simulink model "pfb_fft_d3a"  (R2021a)
settings: Solver=VariableStepAuto  StartTime=0.0  StopTime=100.0  RelTol=1e-3
undefined symbols (not defined in the file): i, pfb_coeff_gen_calc
libraries: xbsIndex_r4 x11529, casper_library_misc x39, casper_library_delays x39, xbsReplacements_r4 x2
(part 52 of 118)

== system pfb_fft_d3a/fft_wideband_real/fft_direct/butterfly2_0/bus_scale/bussify ==
  in1 : Inport
  in2 : Inport  Port=2
  in3 : Inport  Port=3
  in4 : Inport  Port=4
  concatenate : xbsIndex_r4/Concat  num_inputs=4  dbl_ovrd=off  block_type=concat
  reinterpret{1..4} (4 alike) : xbsIndex_r4/Reinterpret  force_arith_type=on  arith_type=Unsigned  force_bin_pt=on  bin_pt=0  block_type=reinterpret
      reinterpret1 settings: infoedit="Changes signal type without altering the binary representation.   You can changed the signal between signed and unsigned, and relocate the binary point.<br><br>Hardware notes: In hardware this block costs nothing.<br><br>Example:  Suppose the input is 6 bits wide, signed, with 2 fractional bits, and the output is forced to unsigned with 0 fractional bits.  Then an input of -2.0 (1110.00 in binary 2's complement) becomes an output of 56 (111000 in binary)."
      reinterpret2 settings: infoedit="Changes signal type without altering the binary representation.   You can changed the signal between signed and unsigned, and relocate the binary point.<br><br>Hardware notes: In hardware this block costs nothing.<br><br>Example:  Suppose the input is 6 bits wide, signed, with 2 fractional bits, and the output is forced to unsigned with 0 fractional bits.  Then an input of -2.0 (1110.00 in binary 2's complement) becomes an output of 56 (111000 in binary)."
  bus_out : Outport  VectorParamsAs1DForOutWhenUnconnected=off
  wires:
  concatenate/1 -> bus_out/1
  in1/1 -> reinterpret1/1
  reinterpret1/1 -> concatenate/1
  in2/1 -> reinterpret2/1
  reinterpret2/1 -> concatenate/2
  in3/1 -> reinterpret3/1
  reinterpret3/1 -> concatenate/3
  in4/1 -> reinterpret4/1
  reinterpret4/1 -> concatenate/4

== system pfb_fft_d3a/fft_wideband_real/fft_direct/butterfly2_0/bus_scale/debus ==
  bus_in : Inport
  reinterpret{1..4} (4 alike) : xbsIndex_r4/Reinterpret  force_arith_type=on  arith_type="Signed  (2's comp)"  force_bin_pt=on  bin_pt=17  block_type=reinterpret
  slice1 : xbsIndex_r4/Slice  nbits=20  boolean_output=off  mode=Upper Bit Location + Width  bit1=-60  base1=MSB of Input  bit0=0  base0=LSB of Input  dbl_ovrd=off  block_type=slice
  slice2 : xbsIndex_r4/Slice  nbits=20  boolean_output=off  mode=Upper Bit Location + Width  bit1=-40  base1=MSB of Input  bit0=0  base0=LSB of Input  dbl_ovrd=off  block_type=slice
  slice3 : xbsIndex_r4/Slice  nbits=20  boolean_output=off  mode=Upper Bit Location + Width  bit1=-20  base1=MSB of Input  bit0=0  base0=LSB of Input  dbl_ovrd=off  block_type=slice
  slice4 : xbsIndex_r4/Slice  nbits=20  boolean_output=off  mode=Upper Bit Location + Width  bit1=0  base1=MSB of Input  bit0=0  base0=LSB of Input  dbl_ovrd=off  block_type=slice
  msb_out4 : Outport
  out3 : Outport  Port=2
  out2 : Outport  Port=3
  lsb_out1 : Outport  Port=4  VectorParamsAs1DForOutWhenUnconnected=off
  wires:
  bus_in/1 -> slice4/1, slice3/1, slice2/1, slice1/1
  slice4/1 -> reinterpret4/1
  reinterpret4/1 -> msb_out4/1
  slice3/1 -> reinterpret3/1
  reinterpret3/1 -> out3/1
  slice2/1 -> reinterpret2/1
  reinterpret2/1 -> out2/1
  slice1/1 -> reinterpret1/1
  reinterpret1/1 -> lsb_out1/1

== system pfb_fft_d3a/fft_wideband_real/fft_direct/butterfly2_0/bus_sub/a_debus ==
  bus_in : Inport
  reinterpret1 : xbsIndex_r4/Reinterpret  force_arith_type=on  arith_type="Signed  (2's comp)"  force_bin_pt=on  bin_pt=17  block_type=reinterpret
  reinterpret2 : xbsIndex_r4/Reinterpret  force_arith_type=on  arith_type="Signed  (2's comp)"  force_bin_pt=on  bin_pt=17  block_type=reinterpret
  slice1 : xbsIndex_r4/Slice  nbits=18  boolean_output=off  mode=Upper Bit Location + Width  bit1=-18  base1=MSB of Input  bit0=0  base0=LSB of Input  dbl_ovrd=off  block_type=slice
  slice2 : xbsIndex_r4/Slice  nbits=18  boolean_output=off  mode=Upper Bit Location + Width  bit1=0  base1=MSB of Input  bit0=0  base0=LSB of Input  dbl_ovrd=off  block_type=slice
  msb_out2 : Outport  VectorParamsAs1DForOutWhenUnconnected=off
  lsb_out1 : Outport  Port=2  VectorParamsAs1DForOutWhenUnconnected=off
  wires:
  bus_in/1 -> slice2/1, slice1/1
  slice2/1 -> reinterpret2/1
  reinterpret2/1 -> msb_out2/1
  slice1/1 -> reinterpret1/1
  reinterpret1/1 -> lsb_out1/1

== system pfb_fft_d3a/fft_wideband_real/fft_direct/butterfly2_0/bus_sub/b_debus ==
  bus_in : Inport
  reinterpret1 : xbsIndex_r4/Reinterpret  force_arith_type=on  arith_type="Signed  (2's comp)"  force_bin_pt=on  bin_pt=17  block_type=reinterpret
  reinterpret2 : xbsIndex_r4/Reinterpret  force_arith_type=on  arith_type="Signed  (2's comp)"  force_bin_pt=on  bin_pt=17  block_type=reinterpret
  slice1 : xbsIndex_r4/Slice  nbits=19  boolean_output=off  mode=Upper Bit Location + Width  bit1=-19  base1=MSB of Input  bit0=0  base0=LSB of Input  dbl_ovrd=off  block_type=slice
  slice2 : xbsIndex_r4/Slice  nbits=19  boolean_output=off  mode=Upper Bit Location + Width  bit1=0  base1=MSB of Input  bit0=0  base0=LSB of Input  dbl_ovrd=off  block_type=slice
  msb_out2 : Outport  VectorParamsAs1DForOutWhenUnconnected=off
  lsb_out1 : Outport  Port=2  VectorParamsAs1DForOutWhenUnconnected=off
  wires:
  bus_in/1 -> slice2/1, slice1/1
  slice2/1 -> reinterpret2/1
  reinterpret2/1 -> msb_out2/1
  slice1/1 -> reinterpret1/1
  reinterpret1/1 -> lsb_out1/1

== system pfb_fft_d3a/fft_wideband_real/fft_direct/butterfly2_0/bus_sub/op_bussify ==
  in1 : Inport
  in2 : Inport  Port=2
  concatenate : xbsIndex_r4/Concat  num_inputs=2  dbl_ovrd=off  block_type=concat
  reinterpret1 : xbsIndex_r4/Reinterpret  force_arith_type=on  arith_type=Unsigned  force_bin_pt=on  bin_pt=0  block_type=reinterpret
      settings: infoedit="Changes signal type without altering the binary representation.   You can changed the signal between signed and unsigned, and relocate the binary point.<br><br>Hardware notes: In hardware this block costs nothing.<br><br>Example:  Suppose the input is 6 bits wide, signed, with 2 fractional bits, and the output is forced to unsigned with 0 fractional bits.  Then an input of -2.0 (1110.00 in binary 2's complement) becomes an output of 56 (111000 in binary)."
  reinterpret2 : xbsIndex_r4/Reinterpret  force_arith_type=on  arith_type=Unsigned  force_bin_pt=on  bin_pt=0  block_type=reinterpret
      settings: infoedit="Changes signal type without altering the binary representation.   You can changed the signal between signed and unsigned, and relocate the binary point.<br><br>Hardware notes: In hardware this block costs nothing.<br><br>Example:  Suppose the input is 6 bits wide, signed, with 2 fractional bits, and the output is forced to unsigned with 0 fractional bits.  Then an input of -2.0 (1110.00 in binary 2's complement) becomes an output of 56 (111000 in binary)."
  bus_out : Outport  VectorParamsAs1DForOutWhenUnconnected=off
  wires:
  concatenate/1 -> bus_out/1
  in1/1 -> reinterpret1/1
  reinterpret1/1 -> concatenate/1
  in2/1 -> reinterpret2/1
  reinterpret2/1 -> concatenate/2

== system pfb_fft_d3a/fft_wideband_real/fft_direct/butterfly2_0/munge/join ==
  in1 : Inport
  in2 : Inport  Port=2
  concatenate : xbsIndex_r4/Concat  num_inputs=2  dbl_ovrd=off  block_type=concat
  reinterpret1 : xbsIndex_r4/Reinterpret  force_arith_type=on  arith_type=Unsigned  force_bin_pt=on  bin_pt=0  block_type=reinterpret
      settings: infoedit="Changes signal type without altering the binary representation.   You can changed the signal between signed and unsigned, and relocate the binary point.<br><br>Hardware notes: In hardware this block costs nothing.<br><br>Example:  Suppose the input is 6 bits wide, signed, with 2 fractional bits, and the output is forced to unsigned with 0 fractional bits.  Then an input of -2.0 (1110.00 in binary 2's complement) becomes an output of 56 (111000 in binary)."
  reinterpret2 : xbsIndex_r4/Reinterpret  force_arith_type=on  arith_type=Unsigned  force_bin_pt=on  bin_pt=0  block_type=reinterpret
      settings: infoedit="Changes signal type without altering the binary representation.   You can changed the signal between signed and unsigned, and relocate the binary point.<br><br>Hardware notes: In hardware this block costs nothing.<br><br>Example:  Suppose the input is 6 bits wide, signed, with 2 fractional bits, and the output is forced to unsigned with 0 fractional bits.  Then an input of -2.0 (1110.00 in binary 2's complement) becomes an output of 56 (111000 in binary)."
  bus_out : Outport  VectorParamsAs1DForOutWhenUnconnected=off
  wires:
  concatenate/1 -> bus_out/1
  in1/1 -> reinterpret1/1
  reinterpret1/1 -> concatenate/1
  in2/1 -> reinterpret2/1
  reinterpret2/1 -> concatenate/2

== system pfb_fft_d3a/fft_wideband_real/fft_direct/butterfly2_0/munge/split ==
  bus_in : Inport
  reinterpret1 : xbsIndex_r4/Reinterpret  force_arith_type=on  arith_type=Unsigned  force_bin_pt=on  bin_pt=0  block_type=reinterpret
  reinterpret2 : xbsIndex_r4/Reinterpret  force_arith_type=on  arith_type=Unsigned  force_bin_pt=on  bin_pt=0  block_type=reinterpret
  slice1 : xbsIndex_r4/Slice  nbits=2  boolean_output=off  mode=Upper Bit Location + Width  bit1=-2  base1=MSB of Input  bit0=0  base0=LSB of Input  dbl_ovrd=off  block_type=slice
  slice2 : xbsIndex_r4/Slice  nbits=2  boolean_output=off  mode=Upper Bit Location + Width  bit1=0  base1=MSB of Input  bit0=0  base0=LSB of Input  dbl_ovrd=off  block_type=slice
  msb_out2 : Outport  VectorParamsAs1DForOutWhenUnconnected=off
  lsb_out1 : Outport  Port=2  VectorParamsAs1DForOutWhenUnconnected=off
  wires:
  bus_in/1 -> slice2/1, slice1/1
  slice2/1 -> reinterpret2/1
  reinterpret2/1 -> msb_out2/1
  slice1/1 -> reinterpret1/1
  reinterpret1/1 -> lsb_out1/1

== system pfb_fft_d3a/fft_wideband_real/fft_direct/butterfly2_0/mux/d_bussify ==
  in1 : Inport
  in2 : Inport  Port=2
  in3 : Inport  Port=3
  in4 : Inport  Port=4
  concatenate : xbsIndex_r4/Concat  num_inputs=4  dbl_ovrd=off  block_type=concat
  reinterpret{1..4} (4 alike) : xbsIndex_r4/Reinterpret  force_arith_type=on  arith_type=Unsigned  force_bin_pt=on  bin_pt=0  block_type=reinterpret
      reinterpret1 settings: infoedit="Changes signal type without altering the binary representation.   You can changed the signal between signed and unsigned, and relocate the binary point.<br><br>Hardware notes: In hardware this block costs nothing.<br><br>Example:  Suppose the input is 6 bits wide, signed, with 2 fractional bits, and the output is forced to unsigned with 0 fractional bits.  Then an input of -2.0 (1110.00 in binary 2's complement) becomes an output of 56 (111000 in binary)."
      reinterpret2 settings: infoedit="Changes signal type without altering the binary representation.   You can changed the signal between signed and unsigned, and relocate the binary point.<br><br>Hardware notes: In hardware this block costs nothing.<br><br>Example:  Suppose the input is 6 bits wide, signed, with 2 fractional bits, and the output is forced to unsigned with 0 fractional bits.  Then an input of -2.0 (1110.00 in binary 2's complement) becomes an output of 56 (111000 in binary)."
  bus_out : Outport  VectorParamsAs1DForOutWhenUnconnected=off
  wires:
  concatenate/1 -> bus_out/1
  in1/1 -> reinterpret1/1
  reinterpret1/1 -> concatenate/1
  in2/1 -> reinterpret2/1
  reinterpret2/1 -> concatenate/2
  in3/1 -> reinterpret3/1
  reinterpret3/1 -> concatenate/3
  in4/1 -> reinterpret4/1
  reinterpret4/1 -> concatenate/4

== system pfb_fft_d3a/fft_wideband_real/fft_direct/butterfly2_0/mux/expand0 ==
  bus_in : Inport
  reinterpret{1..4} (4 alike) : xbsIndex_r4/Reinterpret  force_arith_type=on  arith_type=Unsigned  force_bin_pt=on  bin_pt=0  block_type=reinterpret
  slice1 : xbsIndex_r4/Slice  nbits=21  boolean_output=off  mode=Upper Bit Location + Width  bit1=-63  base1=MSB of Input  bit0=0  base0=LSB of Input  dbl_ovrd=off  block_type=slice
  slice2 : xbsIndex_r4/Slice  nbits=21  boolean_output=off  mode=Upper Bit Location + Width  bit1=-42  base1=MSB of Input  bit0=0  base0=LSB of Input  dbl_ovrd=off  block_type=slice
  slice3 : xbsIndex_r4/Slice  nbits=21  boolean_output=off  mode=Upper Bit Location + Width  bit1=-21  base1=MSB of Input  bit0=0  base0=LSB of Input  dbl_ovrd=off  block_type=slice
  slice4 : xbsIndex_r4/Slice  nbits=21  boolean_output=off  mode=Upper Bit Location + Width  bit1=0  base1=MSB of Input  bit0=0  base0=LSB of Input  dbl_ovrd=off  block_type=slice
  msb_out4 : Outport
  out3 : Outport  Port=2
  out2 : Outport  Port=3
  lsb_out1 : Outport  Port=4  VectorParamsAs1DForOutWhenUnconnected=off
  wires:
  bus_in/1 -> slice4/1, slice3/1, slice2/1, slice1/1
  slice4/1 -> reinterpret4/1
  reinterpret4/1 -> msb_out4/1
  slice3/1 -> reinterpret3/1
  reinterpret3/1 -> out3/1
  slice2/1 -> reinterpret2/1
  reinterpret2/1 -> out2/1
  slice1/1 -> reinterpret1/1
  reinterpret1/1 -> lsb_out1/1

== system pfb_fft_d3a/fft_wideband_real/fft_direct/butterfly2_0/mux/expand1 ==
  bus_in : Inport
  reinterpret{1..4} (4 alike) : xbsIndex_r4/Reinterpret  force_arith_type=on  arith_type=Unsigned  force_bin_pt=on  bin_pt=0  block_type=reinterpret
  slice1 : xbsIndex_r4/Slice  nbits=21  boolean_output=off  mode=Upper Bit Location + Width  bit1=-63  base1=MSB of Input  bit0=0  base0=LSB of Input  dbl_ovrd=off  block_type=slice
  slice2 : xbsIndex_r4/Slice  nbits=21  boolean_output=off  mode=Upper Bit Location + Width  bit1=-42  base1=MSB of Input  bit0=0  base0=LSB of Input  dbl_ovrd=off  block_type=slice
  slice3 : xbsIndex_r4/Slice  nbits=21  boolean_output=off  mode=Upper Bit Location + Width  bit1=-21  base1=MSB of Input  bit0=0  base0=LSB of Input  dbl_ovrd=off  block_type=slice
  slice4 : xbsIndex_r4/Slice  nbits=21  boolean_output=off  mode=Upper Bit Location + Width  bit1=0  base1=MSB of Input  bit0=0  base0=LSB of Input  dbl_ovrd=off  block_type=slice
  msb_out4 : Outport
  out3 : Outport  Port=2
  out2 : Outport  Port=3
  lsb_out1 : Outport  Port=4  VectorParamsAs1DForOutWhenUnconnected=off
  wires:
  bus_in/1 -> slice4/1, slice3/1, slice2/1, slice1/1
  slice4/1 -> reinterpret4/1
  reinterpret4/1 -> msb_out4/1
  slice3/1 -> reinterpret3/1
  reinterpret3/1 -> out3/1
  slice2/1 -> reinterpret2/1
  reinterpret2/1 -> out2/1
  slice1/1 -> reinterpret1/1
  reinterpret1/1 -> lsb_out1/1

== system pfb_fft_d3a/fft_wideband_real/fft_direct/butterfly2_0/mux/sel_expand ==
  bus_in : Inport
  reinterpret{1..4} (4 alike) : xbsIndex_r4/Reinterpret  force_arith_type=on  arith_type=Unsigned  force_bin_pt=on  bin_pt=0  block_type=reinterpret
  slice1 : xbsIndex_r4/Slice  nbits=1  boolean_output=off  mode=Upper Bit Location + Width  bit1=-3  base1=MSB of Input  bit0=0  base0=LSB of Input  dbl_ovrd=off  block_type=slice
  slice2 : xbsIndex_r4/Slice  nbits=1  boolean_output=off  mode=Upper Bit Location + Width  bit1=-2  base1=MSB of Input  bit0=0  base0=LSB of Input  dbl_ovrd=off  block_type=slice
  slice3 : xbsIndex_r4/Slice  nbits=1  boolean_output=off  mode=Upper Bit Location + Width  bit1=-1  base1=MSB of Input  bit0=0  base0=LSB of Input  dbl_ovrd=off  block_type=slice
  slice4 : xbsIndex_r4/Slice  nbits=1  boolean_output=off  mode=Upper Bit Location + Width  bit1=0  base1=MSB of Input  bit0=0  base0=LSB of Input  dbl_ovrd=off  block_type=slice
  msb_out4 : Outport
  out3 : Outport  Port=2
  out2 : Outport  Port=3
  lsb_out1 : Outport  Port=4  VectorParamsAs1DForOutWhenUnconnected=off
  wires:
  bus_in/1 -> slice4/1, slice3/1, slice2/1, slice1/1
  slice4/1 -> reinterpret4/1
  reinterpret4/1 -> msb_out4/1
  slice3/1 -> reinterpret3/1
  reinterpret3/1 -> out3/1
  slice2/1 -> reinterpret2/1
  reinterpret2/1 -> out2/1
  slice1/1 -> reinterpret1/1
  reinterpret1/1 -> lsb_out1/1

== system pfb_fft_d3a/fft_wideband_real/fft_direct/butterfly2_0/shift_replicate/bussify ==
  in1 : Inport
  in2 : Inport  Port=2
  in3 : Inport  Port=3
  in4 : Inport  Port=4
  concatenate : xbsIndex_r4/Concat  num_inputs=4  dbl_ovrd=off  block_type=concat
  reinterpret{1..4} (4 alike) : xbsIndex_r4/Reinterpret  force_arith_type=on  arith_type=Unsigned  force_bin_pt=on  bin_pt=0  block_type=reinterpret
      reinterpret1 settings: infoedit="Changes signal type without altering the binary representation.   You can changed the signal between signed and unsigned, and relocate the binary point.<br><br>Hardware notes: In hardware this block costs nothing.<br><br>Example:  Suppose the input is 6 bits wide, signed, with 2 fractional bits, and the output is forced to unsigned with 0 fractional bits.  Then an input of -2.0 (1110.00 in binary 2's complement) becomes an output of 56 (111000 in binary)."
      reinterpret2 settings: infoedit="Changes signal type without altering the binary representation.   You can changed the signal between signed and unsigned, and relocate the binary point.<br><br>Hardware notes: In hardware this block costs nothing.<br><br>Example:  Suppose the input is 6 bits wide, signed, with 2 fractional bits, and the output is forced to unsigned with 0 fractional bits.  Then an input of -2.0 (1110.00 in binary 2's complement) becomes an output of 56 (111000 in binary)."
  bus_out : Outport  VectorParamsAs1DForOutWhenUnconnected=off
  wires:
  concatenate/1 -> bus_out/1
  in1/1 -> reinterpret1/1
  reinterpret1/1 -> concatenate/1
  in2/1 -> reinterpret2/1
  reinterpret2/1 -> concatenate/2
  in3/1 -> reinterpret3/1
  reinterpret3/1 -> concatenate/3
  in4/1 -> reinterpret4/1
  reinterpret4/1 -> concatenate/4

== system pfb_fft_d3a/fft_wideband_real/fft_direct/butterfly2_0/twiddle/bus_convert ==
  din : Inport
  misci : Inport  Port=2
  bussify : Subsystem  AncestorBlock=casper_library_flow_control/bus_create  mask(bus_create){inputNum=2}
      mask prompts: inputNum "Number of inputs:"
      mask init:
      | bus_create_init(gcb,...
      |     'inputNum', inputNum);
  conv1 : xbsIndex_r4/Convert  gui_display_data_type=Fixed-point  arith_type="Signed  (2's comp)"  n_bits=19  bin_pt=17  float_type=Single  exp_bits=8  fraction_bits=24  quantization="Round  (unbiased: Even Values)"  overflow=Wrap  en=off  latency=1  pipeline=on  dbl_ovrd=off  block_type=convert
  conv2 : xbsIndex_r4/Convert  gui_display_data_type=Fixed-point  arith_type="Signed  (2's comp)"  n_bits=19  bin_pt=17  float_type=Single  exp_bits=8  fraction_bits=24  quantization="Round  (unbiased: Even Values)"  overflow=Wrap  en=off  latency=1  pipeline=on  dbl_ovrd=off  block_type=convert
  debus : Subsystem  AncestorBlock=casper_library_flow_control/bus_expand  mask(bus_expand){mode=divisions of arbitrary size, outputNum=2, outputWidth=[37 37], outputBinaryPt=[34 34], outputArithmeticType=[1 1], show_format=on, outputToWorkspace=off, variablePrefix=, outputToModelAsWell=on}
      mask prompts: outputNum "Number of outputs:"; outputWidth "Output width:"; outputBinaryPt "Output binary point position:"; outputArithmeticType "Output arithmetic type (ufix=0, fix=1, bool=2):"; show_format "Print format string?"; outputToWorkspace "Output to workspace?"; variablePrefix "Variable name prefix:"; outputToModelAsWell "Output to model as well?"
      mask help:
      | Expands a 'bus' made using a bus_create or Xilinx
      | concat block.
      | The input will be divided into the specified number
      | of outputs with the specified arithmetic types.
      | Divisions are made from most significant bit.
      mask init: same as pfb_fft_d3a/fft_wideband_real/fft_biplex_real_4x/pol0_debus
      settings: AttributesFormatString=2 outputs: f37.34,f37.34,
      mask TypeOptions mode: divisions of equal size | divisions of arbitrary size
      mask Callback mode: %bus_expand_callback();
      mask Callback outputWidth: %bus_expand_callback();
      mask Callback outputToWorkspace: %bus_expand_callback();
  dmisc : xbsIndex_r4/Delay  rst=off  infoeditControl=Selection of Reset will increase slice count due to use of real FFs and instead of SRLs  en=off  latency=csp_latency  reg_retiming=on  dbl_ovrd=off  block_type=delay
  dout : Outport
  misco : Outport  Port=2
  wires:
  din/1 -> debus/1(bus_in)
  debus/1(msb_out2) -> conv1/1
  debus/2(lsb_out1) -> conv2/1
  misci/1 -> dmisc/1
  conv1/1 -> bussify/1(in1)
  conv2/1 -> bussify/2(in2)
  bussify/1(bus_out) -> dout/1
  dmisc/1 -> misco/1

== system pfb_fft_d3a/fft_wideband_real/fft_direct/butterfly2_0/twiddle/bus_create ==
  in1 : Inport
  in2 : Inport  Port=2
  in3 : Inport  Port=3
  concatenate : xbsIndex_r4/Concat  num_inputs=3  dbl_ovrd=off  block_type=concat
  reinterpret1 : xbsIndex_r4/Reinterpret  force_arith_type=on  arith_type=Unsigned  force_bin_pt=on  bin_pt=0  block_type=reinterpret
      settings: infoedit="Changes signal type without altering the binary representation.   You can changed the signal between signed and unsigned, and relocate the binary point.<br><br>Hardware notes: In hardware this block costs nothing.<br><br>Example:  Suppose the input is 6 bits wide, signed, with 2 fractional bits, and the output is forced to unsigned with 0 fractional bits.  Then an input of -2.0 (1110.00 in binary 2's complement) becomes an output of 56 (111000 in binary)."
  reinterpret2 : xbsIndex_r4/Reinterpret  force_arith_type=on  arith_type=Unsigned  force_bin_pt=on  bin_pt=0  block_type=reinterpret
      settings: infoedit="Changes signal type without altering the binary representation.   You can changed the signal between signed and unsigned, and relocate the binary point.<br><br>Hardware notes: In hardware this block costs nothing.<br><br>Example:  Suppose the input is 6 bits wide, signed, with 2 fractional bits, and the output is forced to unsigned with 0 fractional bits.  Then an input of -2.0 (1110.00 in binary 2's complement) becomes an output of 56 (111000 in binary)."
  reinterpret3 : xbsIndex_r4/Reinterpret  force_arith_type=on  arith_type=Unsigned  force_bin_pt=on  bin_pt=0  block_type=reinterpret
  bus_out : Outport  VectorParamsAs1DForOutWhenUnconnected=off
  wires:
  concatenate/1 -> bus_out/1
  in1/1 -> reinterpret1/1
  reinterpret1/1 -> concatenate/1
  in2/1 -> reinterpret2/1
  reinterpret2/1 -> concatenate/2
  in3/1 -> reinterpret3/1
  reinterpret3/1 -> concatenate/3

== system pfb_fft_d3a/fft_wideband_real/fft_direct/butterfly2_0/twiddle/bus_expand ==
  bus_in : Inport
  reinterpret1 : xbsIndex_r4/Reinterpret  force_arith_type=on  arith_type=Unsigned  force_bin_pt=on  bin_pt=0  block_type=reinterpret
  reinterpret2 : xbsIndex_r4/Reinterpret  force_arith_type=on  arith_type=Unsigned  force_bin_pt=on  bin_pt=0  block_type=reinterpret
  slice1 : xbsIndex_r4/Slice  nbits=37  boolean_output=off  mode=Upper Bit Location + Width  bit1=-36  base1=MSB of Input  bit0=0  base0=LSB of Input  dbl_ovrd=off  block_type=slice
  slice2 : xbsIndex_r4/Slice  nbits=36  boolean_output=off  mode=Upper Bit Location + Width  bit1=0  base1=MSB of Input  bit0=0  base0=LSB of Input  dbl_ovrd=off  block_type=slice
  msb_out2 : Outport  VectorParamsAs1DForOutWhenUnconnected=off
  lsb_out1 : Outport  Port=2  VectorParamsAs1DForOutWhenUnconnected=off
  wires:
  bus_in/1 -> slice2/1, slice1/1
  slice2/1 -> reinterpret2/1
  reinterpret2/1 -> msb_out2/1
  slice1/1 -> reinterpret1/1
  reinterpret1/1 -> lsb_out1/1

== system pfb_fft_d3a/fft_wideband_real/fft_direct/butterfly2_0/twiddle/bus_expand1 ==
  bus_in : Inport
  reinterpret1 : xbsIndex_r4/Reinterpret  force_arith_type=on  arith_type=Unsigned  force_bin_pt=on  bin_pt=0  block_type=reinterpret
  slice1 : xbsIndex_r4/Slice  nbits=36  boolean_output=off  mode=Upper Bit Location + Width  bit1=-1  base1=MSB of Input  bit0=0  base0=LSB of Input  dbl_ovrd=off  block_type=slice
  slice2 : xbsIndex_r4/Slice  nbits=1  boolean_output=on  mode=Upper Bit Location + Width  bit1=0  base1=MSB of Input  bit0=0  base0=LSB of Input  dbl_ovrd=off  block_type=slice
  msb_out2 : Outport  VectorParamsAs1DForOutWhenUnconnected=off
  lsb_out1 : Outport  Port=2  VectorParamsAs1DForOutWhenUnconnected=off
  wires:
  bus_in/1 -> slice2/1, slice1/1
  slice2/1 -> msb_out2/1
  slice1/1 -> reinterpret1/1
  reinterpret1/1 -> lsb_out1/1

== system pfb_fft_d3a/fft_wideband_real/fft_direct/butterfly2_0/twiddle/bus_mult ==
  a : Inport
  b : Inport  Port=2
  misci : Inport  Port=3
  a*b_bussify : Subsystem  AncestorBlock=casper_library_flow_control/bus_create  mask(bus_create){inputNum=1}
      mask prompts: inputNum "Number of inputs:"
      mask init:
      | bus_create_init(gcb,...
      |     'inputNum', inputNum);
  a_debus : Subsystem  AncestorBlock=casper_library_flow_control/bus_expand  mask(bus_expand){mode=divisions of arbitrary size, outputNum=2, outputWidth=36, outputBinaryPt=0, outputArithmeticType=0, show_format=on, outputToWorkspace=off, variablePrefix=, outputToModelAsWell=on}
      mask prompts: outputNum "Number of outputs:"; outputWidth "Output width:"; outputBinaryPt "Output binary point position:"; outputArithmeticType "Output arithmetic type (ufix=0, fix=1, bool=2):"; show_format "Print format string?"; outputToWorkspace "Output to workspace?"; variablePrefix "Variable name prefix:"; outputToModelAsWell "Output to model as well?"
      mask help:
      | Expands a 'bus' made using a bus_create or Xilinx
      | concat block.
      | The input will be divided into the specified number
      | of outputs with the specified arithmetic types.
      | Divisions are made from most significant bit.
      mask init: same as pfb_fft_d3a/fft_wideband_real/fft_biplex_real_4x/pol0_debus
      settings: AttributesFormatString=1 outputs: uf36.0,
      mask TypeOptions mode: divisions of equal size | divisions of arbitrary size
      mask Callback mode: %bus_expand_callback();
      mask Callback outputWidth: %bus_expand_callback();
      mask Callback outputToWorkspace: %bus_expand_callback();
  b_debus : Subsystem  AncestorBlock=casper_library_flow_control/bus_expand  mask(bus_expand){mode=divisions of arbitrary size, outputNum=2, outputWidth=36, outputBinaryPt=0, outputArithmeticType=0, show_format=on, outputToWorkspace=off, variablePrefix=, outputToModelAsWell=on}
      mask prompts: outputNum "Number of outputs:"; outputWidth "Output width:"; outputBinaryPt "Output binary point position:"; outputArithmeticType "Output arithmetic type (ufix=0, fix=1, bool=2):"; show_format "Print format string?"; outputToWorkspace "Output to workspace?"; variablePrefix "Variable name prefix:"; outputToModelAsWell "Output to model as well?"
      mask help:
      | Expands a 'bus' made using a bus_create or Xilinx
      | concat block.
      | The input will be divided into the specified number
      | of outputs with the specified arithmetic types.
      | Divisions are made from most significant bit.
      mask init: same as pfb_fft_d3a/fft_wideband_real/fft_biplex_real_4x/pol0_debus
      settings: AttributesFormatString=1 outputs: uf36.0,
      mask TypeOptions mode: divisions of equal size | divisions of arbitrary size
      mask Callback mode: %bus_expand_callback();
      mask Callback outputWidth: %bus_expand_callback();
      mask Callback outputToWorkspace: %bus_expand_callback();
  dmisc : xbsIndex_r4/Delay  rst=off  infoeditControl=Selection of Reset will increase slice count due to use of real FFs and instead of SRLs  en=off  latency=mult_latency+add_latency+conv_latency+fan_latency  reg_retiming=on  dbl_ovrd=off  block_type=delay
  mult1 : Subsystem  AncestorBlock=casper_library_multipliers/cmult  mask(cmult){n_bits_a=18, bin_pt_a=17, n_bits_b=18, bin_pt_b=17, n_bits_ab=37, bin_pt_ab=34, quantization=Truncate, overflow=Wrap, conjugated=off, async=off, pipelined_enable=on, floating_point=off, float_type=single, exp_width=8, frac_width=24, in_latency=0, mult_latency=2, add_latency=1, conv_latency=0, pipeline_cmult_en=off, pipeline_latency=0, multiplier_implementation=behavioral HDL}
      mask prompts: n_bits_a "Number of Bits 'a'"; bin_pt_a "Binary Point 'a'"; n_bits_b "Number of Bits 'b'"; bin_pt_b "Binary Point 'b'"; n_bits_ab "Number of Bits 'ab'"; bin_pt_ab "Binary Point 'ab'"; conjugated "Conjugate"; async "asynchronous operation"; pipelined_enable "enable pipeline"; floating_point "floating point"; float_type "float type"; exp_width "exponent width"; frac_width "fraction width"; in_latency "Input latency"; mult_latency "Multiplier Latency"; add_latency "Adder Latency"; conv_latency "Convert latency"; pipeline_cmult_en "Pipeline cmult enable"; pipeline_latency "Pipeline latency"; multiplier_implementation "Multiplier implementation"
      mask help:
      | Multiplies two complex numbers using 4 multipliers and 2 adders.
      | Conjugation is optional.
      mask init: same as pfb_fft_d3a/fft_wideband_real/fft_direct/butterfly0_0/twiddle/bus_mult/mult1
      settings: AttributesFormatString=|
      | 18_17 * 18_17 ==> 37_34
      | Truncate, Wrap
      | Latency=0
      mask TypeOptions quantization: Truncate | Round  (unbiased: +/- Inf) | Round  (unbiased: Even Values)
      mask TypeOptions overflow: Wrap | Saturate | Flag as error
      mask Callback floating_point:
      | onoff = get_param(gcb, 'floating_point');
      | if strcmp(onoff,'on')
      |     enable_fixpt = 'off';
      |     set_param_state(gcb, 'float_type', 'on')
      | 
      |     f_type = get_param(gcb, 'float_type');
      |     if strcmp(f_type,'custom')
      |         set_param_state(gcb, 'exp_width', 'on')
      |         set_param_state(gcb, 'frac_width', 'on')
      |     else
      |         set_param_state(gcb, 'exp_width', 'off')
      |         set_param_state(gcb, 'frac_width', 'off')
      |     end
      | 
      | 
      | else
      |     enable_fixpt = 'on';
      |     set_param_state(gcb, 'float_type', 'off')
      |     set_param_state(gcb, 'exp_width', 'off')
      |     set_param_state(gcb, 'frac_width', 'off')
      | end
      | 
      | 
      | set_param_state(gcb, 'n_bits_a', enable_fixpt)
      | set_param_state(gcb, 'bin_pt_a', enable_fixpt)
      | set_param_state(gcb, 'n_bits_b', enable_fixpt)
      | set_param_state(gcb, 'bin_pt_b', enable_fixpt)
      | set_param_state(gcb, 'n_bits_ab', enable_fixpt)
      | set_param_state(gcb, 'bin_pt_ab', enable_fixpt)
      mask TypeOptions float_type: single | custom
      mask Callback float_type:
      | f_type = get_param(gcb, 'float_type');
      | if strcmp(f_type,'custom')
      |     set_param_state(gcb, 'exp_width', 'on')
      |     set_param_state(gcb, 'frac_width', 'on')
      | else
      |     set_param_state(gcb, 'exp_width', 'off')
      |     set_param_state(gcb, 'frac_width', 'off')
      | end
      mask Callback pipeline_cmult_en:
      | pipeline_en = get_param(gcb, 'pipeline_cmult_en');
      | if strcmp(pipeline_en,'on')
      | 
      |     set_param_state(gcb, 'pipeline_latency', 'on')
      | else
      |     set_param_state(gcb, 'pipeline_latency', 'off')
      | end
      mask TypeOptions multiplier_implementation: behavioral HDL | standard core | embedded multiplier core
      mask DialogControl ParameterTabVar0 Prompt: basic
      mask DialogControl ParameterTabVar01 Prompt: latency
      mask DialogControl ParameterTabVar012 Prompt: implementation
  repa : Subsystem  AncestorBlock=casper_library_bus/bus_replicate  mask(bus_replicate){replication=1, csp_latency=0, misc=off, implementation=core}
      mask prompts: replication "replication factor"; csp_latency "latency"; misc "misc support"; implementation "delay implementation"
      mask help: Output bus formed by replicating input bus a number of times
      mask init:
      | bus_replicate_init(gcb, ...
      |     'replication', replication, ...
      |     'csp_latency', csp_latency, ...
      |     'implementation', implementation, ...
      |     'misc', misc);
      mask TypeOptions implementation: core | behavioral
  repb : Subsystem  AncestorBlock=casper_library_bus/bus_replicate  mask(bus_replicate){replication=1, csp_latency=0, misc=off, implementation=core}
      mask prompts: replication "replication factor"; csp_latency "latency"; misc "misc support"; implementation "delay implementation"
      mask help: Output bus formed by replicating input bus a number of times
      mask init:
      | bus_replicate_init(gcb, ...
      |     'replication', replication, ...
      |     'csp_latency', csp_latency, ...
      |     'implementation', implementation, ...
      |     'misc', misc);
      mask TypeOptions implementation: core | behavioral
  a*b : Outport
  misco : Outport  Port=2
  wires:
  a/1 -> repa/1(in)
  b/1 -> repb/1(in)
  repa/1(out) -> a_debus/1(bus_in)
  repb/1(out) -> b_debus/1(bus_in)
  a_debus/1(msb_lsb_out1) -> mult1/1(a)
  b_debus/1(msb_lsb_out1) -> mult1/2(b)
  misci/1 -> dmisc/1
  mult1/1(ab) -> a*b_bussify/1(in1)
  a*b_bussify/1(bus_out) -> a*b/1
  dmisc/1 -> misco/1

== system pfb_fft_d3a/fft_wideband_real/fft_direct/butterfly2_0/twiddle/coeff_gen ==
  rst : Inport
  misci : Inport  Port=2
  en : xbsIndex_r4/Constant  const=1  gui_display_data_type=Fixed-point  arith_type=Boolean  n_bits=16  bin_pt=14  preci_type=Single  exp_width=8  frac_width=24  explicit_period=on  period=1  equ=P=C  opselect=C  inp2=PCIN>>17  opr=+  inp1=P  carry=CIN  dbl_ovrd=off  block_type=constant
  feedback_osc : Subsystem  Tag=casper:feedback_osc  AncestorBlock=casper_library_downconverter/feedback_osc  mask(feedback_osc){n_bits=coeff_bit_width, n_bits_rotation=n_bits_rotation, phase_initial=0, phase_step_bits=14, phase_steps_bits=11, ref_values_bits=1, bram_latency=2, mult_latency=2, add_latency=1, conv_latency=1, bram=Block RAM, quantization=Round  (unbiased: Even Values)}
      mask prompts: n_bits "output bit resolution"; n_bits_rotation "rotation vector bit resolution"; phase_initial "initial phase ?*(2*pi)"; phase_step_bits "phase step size (2*pi)/2^?"; phase_steps_bits "number phase steps 2^?"; ref_values_bits "number calibration locations (2^?)"; bram_latency "BRAM latency"; mult_latency "multiplier latency"; add_latency "adder latency"; conv_latency "convert latency"; bram "BRAM implementation"; quantization "quantization strategy"
      mask help:
      | A complex exponential generated using an initial vector, complex multiplication
      | to rotate it, and feedback. A lookup table of reference vectors is used
      | to periodically remove accumulated error.
      mask init: same as pfb_fft_d3a/fft_wideband_real/fft_direct/butterfly0_0/twiddle/coeff_gen/feedback_osc
      settings: AttributesFormatString=32 cal vals
      mask TypeOptions bram: Distributed memory | Block RAM
      mask TypeOptions quantization: Truncate | Round  (unbiased: +/- Inf) | Round  (unbiased: Even Values)
  ri_to_c : casper_library_misc/ri_to_c
      settings: SourceProductName=CASPER DSP Blockset
  t0 : Terminator
  t1 : Terminator
  w : Outport
  misco : Outport  Port=2
  wires:
  ri_to_c/1 -> w/1
  en/1 -> feedback_osc/2(en)
  rst/1 -> feedback_osc/1(sync)
  feedback_osc/1(sync_out) -> t0/1
  feedback_osc/4(dvalid) -> t1/1
  feedback_osc/2(cos) -> ri_to_c/1
  feedback_osc/3(-sin) -> ri_to_c/2
  misci/1 -> feedback_osc/3(misci)
  feedback_osc/5(misco) -> misco/1

== system pfb_fft_d3a/fft_wideband_real/fft_direct/butterfly2_1/bus_add/a_debus ==
  bus_in : Inport
  reinterpret1 : xbsIndex_r4/Reinterpret  force_arith_type=on  arith_type="Signed  (2's comp)"  force_bin_pt=on  bin_pt=17  block_type=reinterpret
  reinterpret2 : xbsIndex_r4/Reinterpret  force_arith_type=on  arith_type="Signed  (2's comp)"  force_bin_pt=on  bin_pt=17  block_type=reinterpret
  slice1 : xbsIndex_r4/Slice  nbits=18  boolean_output=off  mode=Upper Bit Location + Width  bit1=-18  base1=MSB of Input  bit0=0  base0=LSB of Input  dbl_ovrd=off  block_type=slice
  slice2 : xbsIndex_r4/Slice  nbits=18  boolean_output=off  mode=Upper Bit Location + Width  bit1=0  base1=MSB of Input  bit0=0  base0=LSB of Input  dbl_ovrd=off  block_type=slice
  msb_out2 : Outport  VectorParamsAs1DForOutWhenUnconnected=off
  lsb_out1 : Outport  Port=2  VectorParamsAs1DForOutWhenUnconnected=off
  wires:
  bus_in/1 -> slice2/1, slice1/1
  slice2/1 -> reinterpret2/1
  reinterpret2/1 -> msb_out2/1
  slice1/1 -> reinterpret1/1
  reinterpret1/1 -> lsb_out1/1

== system pfb_fft_d3a/fft_wideband_real/fft_direct/butterfly2_1/bus_add/b_debus ==
  bus_in : Inport
  reinterpret1 : xbsIndex_r4/Reinterpret  force_arith_type=on  arith_type="Signed  (2's comp)"  force_bin_pt=on  bin_pt=17  block_type=reinterpret
  reinterpret2 : xbsIndex_r4/Reinterpret  force_arith_type=on  arith_type="Signed  (2's comp)"  force_bin_pt=on  bin_pt=17  block_type=reinterpret
  slice1 : xbsIndex_r4/Slice  nbits=19  boolean_output=off  mode=Upper Bit Location + Width  bit1=-19  base1=MSB of Input  bit0=0  base0=LSB of Input  dbl_ovrd=off  block_type=slice
  slice2 : xbsIndex_r4/Slice  nbits=19  boolean_output=off  mode=Upper Bit Location + Width  bit1=0  base1=MSB of Input  bit0=0  base0=LSB of Input  dbl_ovrd=off  block_type=slice
  msb_out2 : Outport  VectorParamsAs1DForOutWhenUnconnected=off
  lsb_out1 : Outport  Port=2  VectorParamsAs1DForOutWhenUnconnected=off
  wires:
  bus_in/1 -> slice2/1, slice1/1
  slice2/1 -> reinterpret2/1
  reinterpret2/1 -> msb_out2/1
  slice1/1 -> reinterpret1/1
  reinterpret1/1 -> lsb_out1/1

== system pfb_fft_d3a/fft_wideband_real/fft_direct/butterfly2_1/bus_add/op_bussify ==
  in1 : Inport
  in2 : Inport  Port=2
  concatenate : xbsIndex_r4/Concat  num_inputs=2  dbl_ovrd=off  block_type=concat
  reinterpret1 : xbsIndex_r4/Reinterpret  force_arith_type=on  arith_type=Unsigned  force_bin_pt=on  bin_pt=0  block_type=reinterpret
      settings: infoedit="Changes signal type without altering the binary representation.   You can changed the signal between signed and unsigned, and relocate the binary point.<br><br>Hardware notes: In hardware this block costs nothing.<br><br>Example:  Suppose the input is 6 bits wide, signed, with 2 fractional bits, and the output is forced to unsigned with 0 fractional bits.  Then an input of -2.0 (1110.00 in binary 2's complement) becomes an output of 56 (111000 in binary)."
  reinterpret2 : xbsIndex_r4/Reinterpret  force_arith_type=on  arith_type=Unsigned  force_bin_pt=on  bin_pt=0  block_type=reinterpret
      settings: infoedit="Changes signal type without altering the binary representation.   You can changed the signal between signed and unsigned, and relocate the binary point.<br><br>Hardware notes: In hardware this block costs nothing.<br><br>Example:  Suppose the input is 6 bits wide, signed, with 2 fractional bits, and the output is forced to unsigned with 0 fractional bits.  Then an input of -2.0 (1110.00 in binary 2's complement) becomes an output of 56 (111000 in binary)."
  bus_out : Outport  VectorParamsAs1DForOutWhenUnconnected=off
  wires:
  concatenate/1 -> bus_out/1
  in1/1 -> reinterpret1/1
  reinterpret1/1 -> concatenate/1
  in2/1 -> reinterpret2/1
  reinterpret2/1 -> concatenate/2

== system pfb_fft_d3a/fft_wideband_real/fft_direct/butterfly2_1/bus_convert/bussify ==
  in1 : Inport
  in2 : Inport  Port=2
  in3 : Inport  Port=3
  in4 : Inport  Port=4
  concatenate : xbsIndex_r4/Concat  num_inputs=4  dbl_ovrd=off  block_type=concat
  reinterpret{1..4} (4 alike) : xbsIndex_r4/Reinterpret  force_arith_type=on  arith_type=Unsigned  force_bin_pt=on  bin_pt=0  block_type=reinterpret
      reinterpret1 settings: infoedit="Changes signal type without altering the binary representation.   You can changed the signal between signed and unsigned, and relocate the binary point.<br><br>Hardware notes: In hardware this block costs nothing.<br><br>Example:  Suppose the input is 6 bits wide, signed, with 2 fractional bits, and the output is forced to unsigned with 0 fractional bits.  Then an input of -2.0 (1110.00 in binary 2's complement) becomes an output of 56 (111000 in binary)."
      reinterpret2 settings: infoedit="Changes signal type without altering the binary representation.   You can changed the signal between signed and unsigned, and relocate the binary point.<br><br>Hardware notes: In hardware this block costs nothing.<br><br>Example:  Suppose the input is 6 bits wide, signed, with 2 fractional bits, and the output is forced to unsigned with 0 fractional bits.  Then an input of -2.0 (1110.00 in binary 2's complement) becomes an output of 56 (111000 in binary)."
  bus_out : Outport  VectorParamsAs1DForOutWhenUnconnected=off
  wires:
  concatenate/1 -> bus_out/1
  in1/1 -> reinterpret1/1
  reinterpret1/1 -> concatenate/1
  in2/1 -> reinterpret2/1
  reinterpret2/1 -> concatenate/2
  in3/1 -> reinterpret3/1
  reinterpret3/1 -> concatenate/3
  in4/1 -> reinterpret4/1
  reinterpret4/1 -> concatenate/4

== system pfb_fft_d3a/fft_wideband_real/fft_direct/butterfly2_1/bus_convert/conv1 ==
  din : Inport
  all_0s : xbsIndex_r4/Logical  logical_function=NAND  inputs=3  en=off  latency=1  precision=Full  arith_type=Unsigned  n_bits=16  bin_pt=0  align_bp=on  dbl_ovrd=off  block_type=logical
  all_1s : xbsIndex_r4/Logical  logical_function=NAND  inputs=3  en=off  latency=1  precision=Full  arith_type=Unsigned  n_bits=16  bin_pt=0  align_bp=on  dbl_ovrd=off  block_type=logical
  and : xbsIndex_r4/Logical  logical_function=AND  inputs=2  en=off  latency=0  precision=Full  arith_type=Unsigned  n_bits=16  bin_pt=0  align_bp=on  dbl_ovrd=off  block_type=logical
  convert : xbsIndex_r4/Convert  gui_display_data_type=Fixed-point  arith_type="Signed  (2's comp)"  n_bits=bit_width_o  bin_pt=binary_point_o  float_type=Single  exp_bits=8  fraction_bits=24  quantization="Round  (unbiased: Even Values)"  overflow=Wrap  en=off  latency=csp_latency  pipeline=on  dbl_ovrd=off  block_type=convert
  invert1 : xbsIndex_r4/Inverter  en=off  latency=0  dbl_ovrd=off  block_type=inv
  invert2 : xbsIndex_r4/Inverter  en=off  latency=0  dbl_ovrd=off  block_type=inv
  invert3 : xbsIndex_r4/Inverter  en=off  latency=0  dbl_ovrd=off  block_type=inv
  slice1 : xbsIndex_r4/Slice  nbits=1  boolean_output=on  mode=Upper Bit Location + Width  bit1=0  base1=MSB of Input  bit0=0  base0=LSB of Input  dbl_ovrd=off  block_type=slice
  slice2 : xbsIndex_r4/Slice  nbits=1  boolean_output=on  mode=Upper Bit Location + Width  bit1=-1  base1=MSB of Input  bit0=0  base0=LSB of Input  dbl_ovrd=off  block_type=slice
  slice3 : xbsIndex_r4/Slice  nbits=1  boolean_output=on  mode=Upper Bit Location + Width  bit1=-2  base1=MSB of Input  bit0=0  base0=LSB of Input  dbl_ovrd=off  block_type=slice
  dout : Outport
  of : Outport  Port=2
  wires:
  din/1 -> convert/1, slice1/1, slice2/1, slice3/1
  convert/1 -> dout/1
  slice1/1 -> all_1s/1, invert1/1
  invert1/1 -> all_0s/1
  slice2/1 -> all_1s/2, invert2/1
  invert2/1 -> all_0s/2
  slice3/1 -> all_1s/3, invert3/1
  invert3/1 -> all_0s/3
  all_0s/1 -> and/1
  all_1s/1 -> and/2
  and/1 -> of/1

== system pfb_fft_d3a/fft_wideband_real/fft_direct/butterfly2_1/bus_convert/conv2 ==
  din : Inport
  all_0s : xbsIndex_r4/Logical  logical_function=NAND  inputs=3  en=off  latency=1  precision=Full  arith_type=Unsigned  n_bits=16  bin_pt=0  align_bp=on  dbl_ovrd=off  block_type=logical
  all_1s : xbsIndex_r4/Logical  logical_function=NAND  inputs=3  en=off  latency=1  precision=Full  arith_type=Unsigned  n_bits=16  bin_pt=0  align_bp=on  dbl_ovrd=off  block_type=logical
  and : xbsIndex_r4/Logical  logical_function=AND  inputs=2  en=off  latency=0  precision=Full  arith_type=Unsigned  n_bits=16  bin_pt=0  align_bp=on  dbl_ovrd=off  block_type=logical
  convert : xbsIndex_r4/Convert  gui_display_data_type=Fixed-point  arith_type="Signed  (2's comp)"  n_bits=bit_width_o  bin_pt=binary_point_o  float_type=Single  exp_bits=8  fraction_bits=24  quantization="Round  (unbiased: Even Values)"  overflow=Wrap  en=off  latency=csp_latency  pipeline=on  dbl_ovrd=off  block_type=convert
  invert1 : xbsIndex_r4/Inverter  en=off  latency=0  dbl_ovrd=off  block_type=inv
  invert2 : xbsIndex_r4/Inverter  en=off  latency=0  dbl_ovrd=off  block_type=inv
  invert3 : xbsIndex_r4/Inverter  en=off  latency=0  dbl_ovrd=off  block_type=inv
  slice1 : xbsIndex_r4/Slice  nbits=1  boolean_output=on  mode=Upper Bit Location + Width  bit1=0  base1=MSB of Input  bit0=0  base0=LSB of Input  dbl_ovrd=off  block_type=slice
  slice2 : xbsIndex_r4/Slice  nbits=1  boolean_output=on  mode=Upper Bit Location + Width  bit1=-1  base1=MSB of Input  bit0=0  base0=LSB of Input  dbl_ovrd=off  block_type=slice
  slice3 : xbsIndex_r4/Slice  nbits=1  boolean_output=on  mode=Upper Bit Location + Width  bit1=-2  base1=MSB of Input  bit0=0  base0=LSB of Input  dbl_ovrd=off  block_type=slice
  dout : Outport
  of : Outport  Port=2
  wires:
  din/1 -> convert/1, slice1/1, slice2/1, slice3/1
  convert/1 -> dout/1
  slice1/1 -> all_1s/1, invert1/1
  invert1/1 -> all_0s/1
  slice2/1 -> all_1s/2, invert2/1
  invert2/1 -> all_0s/2
  slice3/1 -> all_1s/3, invert3/1
  invert3/1 -> all_0s/3
  all_0s/1 -> and/1
  all_1s/1 -> and/2
  and/1 -> of/1

== system pfb_fft_d3a/fft_wideband_real/fft_direct/butterfly2_1/bus_convert/conv3 ==
  din : Inport
  all_0s : xbsIndex_r4/Logical  logical_function=NAND  inputs=3  en=off  latency=1  precision=Full  arith_type=Unsigned  n_bits=16  bin_pt=0  align_bp=on  dbl_ovrd=off  block_type=logical
  all_1s : xbsIndex_r4/Logical  logical_function=NAND  inputs=3  en=off  latency=1  precision=Full  arith_type=Unsigned  n_bits=16  bin_pt=0  align_bp=on  dbl_ovrd=off  block_type=logical
  and : xbsIndex_r4/Logical  logical_function=AND  inputs=2  en=off  latency=0  precision=Full  arith_type=Unsigned  n_bits=16  bin_pt=0  align_bp=on  dbl_ovrd=off  block_type=logical
  convert : xbsIndex_r4/Convert  gui_display_data_type=Fixed-point  arith_type="Signed  (2's comp)"  n_bits=bit_width_o  bin_pt=binary_point_o  float_type=Single  exp_bits=8  fraction_bits=24  quantization="Round  (unbiased: Even Values)"  overflow=Wrap  en=off  latency=csp_latency  pipeline=on  dbl_ovrd=off  block_type=convert
  invert1 : xbsIndex_r4/Inverter  en=off  latency=0  dbl_ovrd=off  block_type=inv
  invert2 : xbsIndex_r4/Inverter  en=off  latency=0  dbl_ovrd=off  block_type=inv
  invert3 : xbsIndex_r4/Inverter  en=off  latency=0  dbl_ovrd=off  block_type=inv
  slice1 : xbsIndex_r4/Slice  nbits=1  boolean_output=on  mode=Upper Bit Location + Width  bit1=0  base1=MSB of Input  bit0=0  base0=LSB of Input  dbl_ovrd=off  block_type=slice
  slice2 : xbsIndex_r4/Slice  nbits=1  boolean_output=on  mode=Upper Bit Location + Width  bit1=-1  base1=MSB of Input  bit0=0  base0=LSB of Input  dbl_ovrd=off  block_type=slice
  slice3 : xbsIndex_r4/Slice  nbits=1  boolean_output=on  mode=Upper Bit Location + Width  bit1=-2  base1=MSB of Input  bit0=0  base0=LSB of Input  dbl_ovrd=off  block_type=slice
  dout : Outport
  of : Outport  Port=2
  wires:
  din/1 -> convert/1, slice1/1, slice2/1, slice3/1
  convert/1 -> dout/1
  slice1/1 -> all_1s/1, invert1/1
  invert1/1 -> all_0s/1
  slice2/1 -> all_1s/2, invert2/1
  invert2/1 -> all_0s/2
  slice3/1 -> all_1s/3, invert3/1
  invert3/1 -> all_0s/3
  all_0s/1 -> and/1
  all_1s/1 -> and/2
  and/1 -> of/1

== system pfb_fft_d3a/fft_wideband_real/fft_direct/butterfly2_1/bus_convert/conv4 ==
  din : Inport
  all_0s : xbsIndex_r4/Logical  logical_function=NAND  inputs=3  en=off  latency=1  precision=Full  arith_type=Unsigned  n_bits=16  bin_pt=0  align_bp=on  dbl_ovrd=off  block_type=logical
  all_1s : xbsIndex_r4/Logical  logical_function=NAND  inputs=3  en=off  latency=1  precision=Full  arith_type=Unsigned  n_bits=16  bin_pt=0  align_bp=on  dbl_ovrd=off  block_type=logical
  and : xbsIndex_r4/Logical  logical_function=AND  inputs=2  en=off  latency=0  precision=Full  arith_type=Unsigned  n_bits=16  bin_pt=0  align_bp=on  dbl_ovrd=off  block_type=logical
  convert : xbsIndex_r4/Convert  gui_display_data_type=Fixed-point  arith_type="Signed  (2's comp)"  n_bits=bit_width_o  bin_pt=binary_point_o  float_type=Single  exp_bits=8  fraction_bits=24  quantization="Round  (unbiased: Even Values)"  overflow=Wrap  en=off  latency=csp_latency  pipeline=on  dbl_ovrd=off  block_type=convert
  invert1 : xbsIndex_r4/Inverter  en=off  latency=0  dbl_ovrd=off  block_type=inv
  invert2 : xbsIndex_r4/Inverter  en=off  latency=0  dbl_ovrd=off  block_type=inv
  invert3 : xbsIndex_r4/Inverter  en=off  latency=0  dbl_ovrd=off  block_type=inv
  slice1 : xbsIndex_r4/Slice  nbits=1  boolean_output=on  mode=Upper Bit Location + Width  bit1=0  base1=MSB of Input  bit0=0  base0=LSB of Input  dbl_ovrd=off  block_type=slice
  slice2 : xbsIndex_r4/Slice  nbits=1  boolean_output=on  mode=Upper Bit Location + Width  bit1=-1  base1=MSB of Input  bit0=0  base0=LSB of Input  dbl_ovrd=off  block_type=slice
  slice3 : xbsIndex_r4/Slice  nbits=1  boolean_output=on  mode=Upper Bit Location + Width  bit1=-2  base1=MSB of Input  bit0=0  base0=LSB of Input  dbl_ovrd=off  block_type=slice
  dout : Outport
  of : Outport  Port=2
  wires:
  din/1 -> convert/1, slice1/1, slice2/1, slice3/1
  convert/1 -> dout/1
  slice1/1 -> all_1s/1, invert1/1
  invert1/1 -> all_0s/1
  slice2/1 -> all_1s/2, invert2/1
  invert2/1 -> all_0s/2
  slice3/1 -> all_1s/3, invert3/1
  invert3/1 -> all_0s/3
  all_0s/1 -> and/1
  all_1s/1 -> and/2
  and/1 -> of/1
